simulink library "controls_element_lib"  (R2018b)
settings: Solver=VariableStepAuto  StartTime=0.0  StopTime=10.0  RelTol=1e-3
undefined symbols (not defined in the file): F_NOM, I_INV_BASE, j, P_INV_NOM, S_INV_NOM, S_NOM, S_PLANT, VHV_NOM, VLL_INV_NOM, VLL_NOM, Z_INV_BASE
libraries: simulink x20, $bdroot x5
(part 2 of 2)

== system controls_element_lib/acMonitor_A/SOGI ==
  in : Inport
  fnom : Inport  Port=2
  2pi : Gain  Gain=2*pi
  Integrator2 : Integrator
  Integrator3 : Integrator
  Product : Product
  Product1 : Product
  Sum4 : Sum  Inputs=|+-
  Sum5 : Sum  Inputs=|+-
  alpha : Gain  Gain=1 / sqrt(2)
  notch : Outport
  bpf : Outport  Port=2
  wires:
  in/1 -> Sum5/1
  fnom/1 -> 2pi/1
  Integrator2/1 -> Product1/1, Sum5/2, bpf/1
  alpha/1 -> Sum4/1
  Sum5/1 -> alpha/1, notch/1
  Sum4/1 -> Product/1
  Integrator3/1 -> Sum4/2
  2pi/1 -> Product1/2, Product/2
  Product/1 -> Integrator2/1
  Product1/1 -> Integrator3/1

== system controls_element_lib/circuitControls_B (SST)/virtual damper ==
  v : Inport
  1/tau_damp : Gain  Gain=1/250e-6
  Integrator : Integrator
  Sum : Sum  Inputs=|+-
  g_damp : Gain  Gain=1/(0.8*Z_INV_BASE)
  i_damp : Outport
  wires:
  1/tau_damp/1 -> Integrator/1
  Integrator/1 -> Sum/2
  v/1 -> Sum/1
  Sum/1 -> 1/tau_damp/1, g_damp/1
  g_damp/1 -> i_damp/1

== system controls_element_lib/circuit_controls_A/LPF ==
  1 : Inport
  Gain2 : Gain  Gain=1/20e-6
  Integrator : Integrator
  Sum4 : Sum  Inputs=|+-
  Out1 : Outport
  wires:
  Sum4/1 -> Gain2/1
  1/1 -> Sum4/1
  Integrator/1 -> Out1/1, Sum4/2
  Gain2/1 -> Integrator/1

== system controls_element_lib/circuit_controls_A/LPF1 ==
  1 : Inport
  Gain2 : Gain  Gain=1/20e-6
  Integrator : Integrator
  Sum4 : Sum  Inputs=|+-
  Out1 : Outport
  wires:
  Sum4/1 -> Gain2/1
  1/1 -> Sum4/1
  Integrator/1 -> Out1/1, Sum4/2
  Gain2/1 -> Integrator/1

== system controls_element_lib/circuit_controls_A/LPF2 ==
  1 : Inport
  Gain2 : Gain  Gain=1/20e-6
  Integrator : Integrator
  Sum4 : Sum  Inputs=|+-
  Out1 : Outport
  wires:
  Gain2/1 -> Integrator/1
  Integrator/1 -> Sum4/2, Out1/1
  1/1 -> Sum4/1
  Sum4/1 -> Gain2/1

== system controls_element_lib/circuit_controls_A/virtual damper ==
  v : Inport
  1/tau_damp : Gain  Gain=1/250e-6
  Integrator : Integrator
  Sum : Sum  Inputs=|+-
  g_damp : Gain  Gain=1/(0.8*Z_INV_BASE)
  i_damp : Outport
  wires:
  1/tau_damp/1 -> Integrator/1
  Integrator/1 -> Sum/2
  v/1 -> Sum/1
  Sum/1 -> 1/tau_damp/1, g_damp/1
  g_damp/1 -> i_damp/1

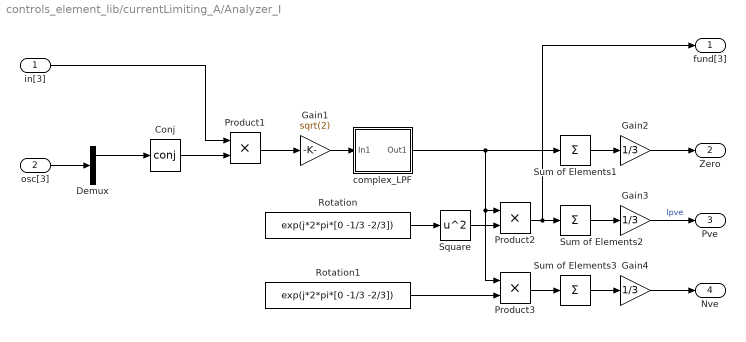
== system controls_element_lib/currentLimiting_A/Analyzer_I ==
  in[3] : Inport
  osc[3] : Inport  Port=2
  Conj : Math  Operator=conj  SaturateOnIntegerOverflow=on
  Demux : Demux  Outputs=3
  Gain1 : Gain  Gain=sqrt(2)
  Gain2 : Gain  Gain=1/3
  Gain3 : Gain  Gain=1/3
  Gain4 : Gain  Gain=1/3
  Product1 : Product
  Product2 : Product
  Product3 : Product
  Rotation : Constant  Value=exp(j*2*pi*[0 -1/3 -2/3])
  Rotation1 : Constant  Value=exp(j*2*pi*[0 -1/3 -2/3])
  Square : Math  Operator=square  SaturateOnIntegerOverflow=on
  Sum of Elements1 : Sum  Inputs=+
  Sum of Elements2 : Sum  Inputs=+
  Sum of Elements3 : Sum  Inputs=+
  complex_LPF : Subsystem  mask{tau=0.02}
      mask prompts: tau "Time constant"
  fund[3] : Outport
  Zero : Outport  Port=2
  Pve : Outport  Port=3
  Nve : Outport  Port=4
  wires:
  in[3]/1 -> Product1/1
  Gain2/1 -> Zero/1
  Gain3/1 -> Pve/1  "Ipve"
  osc[3]/1 -> Demux/1
  Sum of Elements3/1 -> Gain4/1
  Square/1 -> Product2/2
  Sum of Elements1/1 -> Gain2/1
  Conj/1 -> Product1/2
  Sum of Elements2/1 -> Gain3/1
  Rotation1/1 -> Product3/2
  Rotation/1 -> Square/1
  Demux/1 -> Conj/1
  Gain1/1 -> complex_LPF/1(In1)
  Product3/1 -> Sum of Elements3/1
  Product1/1 -> Gain1/1
  complex_LPF/1(Out1) -> Sum of Elements1/1, Product2/1, Product3/1
  Product2/1 -> Sum of Elements2/1, fund[3]/1
  Gain4/1 -> Nve/1

== system controls_element_lib/currentLimiting_A/excess_sink ==
  I_total[3] : Inport
  osc[3] : Inport  Port=2
  Irms_limit : Inport  Port=3
  Complex to Real-Imag : ComplexToRealImag
  Product3 : Product
  RMS Limiter : Subsystem
  Sum : Sum  Inputs=|-+
  sqrt(2) : Gain  Gain=sqrt(2)
  i_excess[3] : Outport
  wires:
  sqrt(2)/1 -> Product3/2
  Product3/1 -> Complex to Real-Imag/1
  I_total[3]/1 -> RMS Limiter/2(I[3]), Sum/2
  Sum/1 -> Product3/1  "Iexcess[3]"
  Complex to Real-Imag/1 -> i_excess[3]/1
  osc[3]/1 -> sqrt(2)/1
  Irms_limit/1 -> RMS Limiter/1(limit)
  RMS Limiter/1(I_limited[3]) -> Sum/1

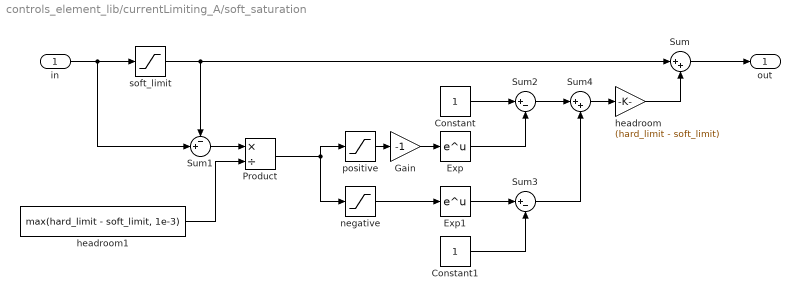
== system controls_element_lib/currentLimiting_A/soft_saturation ==
  in : Inport
  Constant : Constant
  Constant1 : Constant
  Exp : Math  SaturateOnIntegerOverflow=on
  Exp1 : Math  SaturateOnIntegerOverflow=on
  Gain : Gain  Gain=-1
  Product : Product  Inputs=*/
  Sum : Sum  Inputs=|++
  Sum1 : Sum  Inputs=-+|
  Sum2 : Sum  Inputs=|+-
  Sum3 : Sum  Inputs=|+-
  Sum4 : Sum  Inputs=|++
  headroom : Gain  Gain=(hard_limit - soft_limit)
  headroom1 : Constant  Value=max(hard_limit - soft_limit, 1e-3)
  negative : Saturate  UpperLimit=0  LowerLimit=-inf
  positive : Saturate  UpperLimit=inf  LowerLimit=0
  soft_limit : Saturate  UpperLimit=soft_limit  LowerLimit=-soft_limit
  out : Outport
  wires:
  Constant/1 -> Sum2/1
  Product/1 -> negative/1, positive/1
  Constant1/1 -> Sum3/2
  negative/1 -> Exp1/1
  Sum3/1 -> Sum4/2
  soft_limit/1 -> Sum/1, Sum1/1
  Sum/1 -> out/1
  Exp1/1 -> Sum3/1
  in/1 -> Sum1/2, soft_limit/1
  positive/1 -> Gain/1
  Exp/1 -> Sum2/2
  headroom/1 -> Sum/2
  Gain/1 -> Exp/1
  Sum4/1 -> headroom/1
  Sum2/1 -> Sum4/1
  Sum1/1 -> Product/1
  headroom1/1 -> Product/2

== system controls_element_lib/currentLimiting_B/RMS_Analyzer ==
  in : Inport
  Gain : Gain  Gain=1/0.02
  Integrator : Integrator
  Sqrt : Sqrt  SaturateOnIntegerOverflow=on
  Square : Math  Operator=square  SaturateOnIntegerOverflow=on
  Sum : Sum  Inputs=|+-
  RMS : Outport
  wires:
  Sqrt/1 -> RMS/1
  Integrator/1 -> Sqrt/1, Sum/2
  Sum/1 -> Gain/1
  Gain/1 -> Integrator/1
  in/1 -> Square/1
  Square/1 -> Sum/1

== system controls_element_lib/currentLimiting_B/SOGI_BPF ==
  in : Inport
  f : Inport  Port=2
  Gain : Gain
  Gain2 : Gain  Gain=2*pi
  Integrator : Integrator
  Integrator1 : Integrator
  Product : Product
  Product2 : Product
  Sum : Sum  Inputs=|+-
  Sum1 : Sum  Inputs=|+-
  bpf : Outport
  wires:
  Product2/1 -> Sum/2
  Sum/1 -> Product/1
  Gain2/1 -> Product/2, Product2/2
  Integrator/1 -> bpf/1, Gain/1, Integrator1/1
  Sum1/1 -> Sum/1
  Gain/1 -> Sum1/2
  Integrator1/1 -> Product2/1
  Product/1 -> Integrator/1
  in/1 -> Sum1/1
  f/1 -> Gain2/1

== system controls_element_lib/currentLimiting_B/estimate_excess ==
  Ilimit : Inport
  I[3] : Inport  Port=2
  Abs1 : Abs
  Constant : Constant
  Max : MinMax  Function=max
  Min : MinMax  Function=max  Inputs=2
  Product1 : Product  Inputs=*/
  Sum : Sum  Inputs=|+-
  excess_fraction : Outport
  wires:
  Min/1 -> Product1/2
  I[3]/1 -> Abs1/1
  Abs1/1 -> Max/1
  Ilimit/1 -> Min/1, Product1/1  "Irms_limit"
  Max/1 -> Min/2  "max_Iph"
  Product1/1 -> Sum/2  "scale_factor"
  Constant/1 -> Sum/1
  Sum/1 -> excess_fraction/1

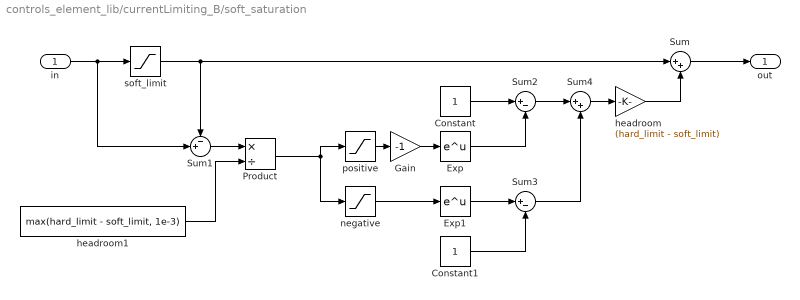
== system controls_element_lib/currentLimiting_B/soft_saturation ==
  in : Inport
  Constant : Constant
  Constant1 : Constant
  Exp : Math  SaturateOnIntegerOverflow=on
  Exp1 : Math  SaturateOnIntegerOverflow=on
  Gain : Gain  Gain=-1
  Product : Product  Inputs=*/
  Sum : Sum  Inputs=|++
  Sum1 : Sum  Inputs=-+|
  Sum2 : Sum  Inputs=|+-
  Sum3 : Sum  Inputs=|+-
  Sum4 : Sum  Inputs=|++
  headroom : Gain  Gain=(hard_limit - soft_limit)
  headroom1 : Constant  Value=max(hard_limit - soft_limit, 1e-3)
  negative : Saturate  UpperLimit=0  LowerLimit=-inf
  positive : Saturate  UpperLimit=inf  LowerLimit=0
  soft_limit : Saturate  UpperLimit=soft_limit  LowerLimit=-soft_limit
  out : Outport
  wires:
  Constant/1 -> Sum2/1
  Product/1 -> negative/1, positive/1
  Constant1/1 -> Sum3/2
  negative/1 -> Exp1/1
  Sum3/1 -> Sum4/2
  soft_limit/1 -> Sum/1, Sum1/1
  Sum/1 -> out/1
  Exp1/1 -> Sum3/1
  in/1 -> Sum1/2, soft_limit/1
  positive/1 -> Gain/1
  Exp/1 -> Sum2/2
  headroom/1 -> Sum/2
  Gain/1 -> Exp/1
  Sum4/1 -> headroom/1
  Sum2/1 -> Sum4/1
  Sum1/1 -> Product/1
  headroom1/1 -> Product/2

== system controls_element_lib/currentSource_A/current_modulator ==
  I_cmd : Inport
  osc : Inport  Port=2
  Complex to Real-Imag : ComplexToRealImag
  Complex to Real-Imag1 : ComplexToRealImag
  Gain : Gain  Gain=sqrt(2)
  Product1 : Product
  Product2 : Product
  Sum1 : Sum  Inputs=|+-
  i_ref : Outport
  wires:
  Complex to Real-Imag1/2 -> Product1/1
  Complex to Real-Imag1/1 -> Product2/1
  I_cmd/1 -> Complex to Real-Imag1/1
  Product1/1 -> Sum1/2
  Complex to Real-Imag/2 -> Product1/2
  Gain/1 -> Complex to Real-Imag/1
  Sum1/1 -> i_ref/1  "i"
  Product2/1 -> Sum1/1
  Complex to Real-Imag/1 -> Product2/2
  osc/1 -> Gain/1

== system controls_element_lib/dcVoltageRegulator_A/SOGI ==
  in : Inport
  fnom : Inport  Port=2
  2pi : Gain  Gain=2*pi
  Integrator2 : Integrator
  Integrator3 : Integrator
  Product : Product
  Product1 : Product
  Sum4 : Sum  Inputs=|+-
  Sum5 : Sum  Inputs=|+-
  alpha : Gain  Gain=1/sqrt(2)
  notch : Outport
  bpf : Outport  Port=2
  wires:
  in/1 -> Sum5/1
  fnom/1 -> 2pi/1
  Integrator2/1 -> Product1/1, Sum5/2, bpf/1
  alpha/1 -> Sum4/1
  Sum5/1 -> alpha/1, notch/1
  Sum4/1 -> Product/1
  Integrator3/1 -> Sum4/2
  2pi/1 -> Product1/2, Product/2
  Product/1 -> Integrator2/1
  Product1/1 -> Integrator3/1

== system controls_element_lib/machineModel_A/excitation ==
  note: This limit is needed to avoid excessive currents during blackstart that cause windup in current limiting logic.. It results in a linear ramp of voltage during blackstart
  VRef : Inport
  osc[3] : Inport  Port=2
  Vd : Inport  Port=3
  Complex to Real-Imag : ComplexToRealImag
  Gain2 : Gain  Gain=1/sqrt(3)
  LPF : TransferFcn  Denominator=[1/wExciter 1]
  Min : MinMax  Inputs=2
  Product1 : Product
  Saturation1 : Saturate  UpperLimit=1.1*VllRated  LowerLimit=0.9*VllRated
  Sum : Sum  Inputs=++|
  assymmetric filter1 : Subsystem
  sqrt(2) : Gain  Gain=sqrt(2)
  voltage_headroom : Constant  Value=0.3*VllRated
  v_emf : Outport
  wires:
  Vd/1 -> assymmetric filter1/1(in)  "Vd"
  assymmetric filter1/1(out) -> Sum/2  "Vd_conditioned"
  Product1/1 -> sqrt(2)/1
  Complex to Real-Imag/1 -> Product1/2
  osc[3]/1 -> Complex to Real-Imag/1
  Gain2/1 -> Product1/1  "Vref_LN"
  sqrt(2)/1 -> v_emf/1
  VRef/1 -> Saturation1/1  "VRef"
  Min/1 -> LPF/1
  LPF/1 -> Gain2/1  "Vref_LL"
  voltage_headroom/1 -> Sum/1
  Saturation1/1 -> Min/1
  Sum/1 -> Min/2

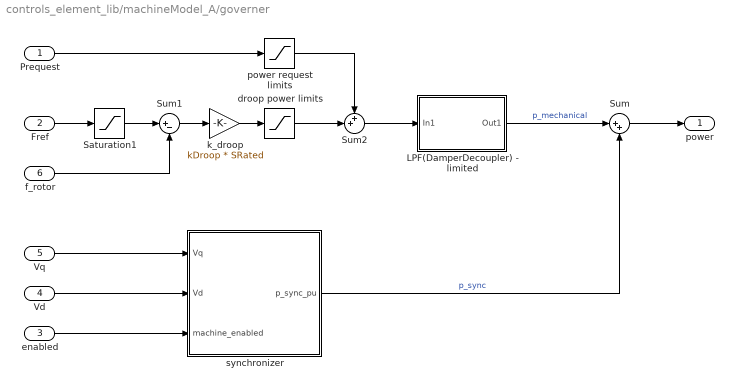
== system controls_element_lib/machineModel_A/governer ==
  Prequest : Inport
  Fref : Inport  Port=2
  enabled : Inport  Port=3
  Vd : Inport  Port=4
  Vq : Inport  Port=5
  f_rotor : Inport  Port=6
  LPF(DamperDecoupler) - limited : Subsystem
  Saturation1 : Saturate  UpperLimit=nominalFrequency+1  LowerLimit=nominalFrequency-1
  Sum : Sum  Inputs=|++
  Sum1 : Sum  Inputs=|+-
  Sum2 : Sum  Inputs=++|
  droop power limits : Saturate  UpperLimit=SRated  LowerLimit=-SRated
  k_droop : Gain  Gain=kDroop * SRated
  power request limits : Saturate  UpperLimit=SRated  LowerLimit=-SRated
  synchronizer : Subsystem
  power : Outport
  wires:
  Vd/1 -> synchronizer/2(Vd)
  Sum1/1 -> k_droop/1
  Sum/1 -> power/1
  Fref/1 -> Saturation1/1
  f_rotor/1 -> Sum1/2
  Saturation1/1 -> Sum1/1
  LPF(DamperDecoupler) - limited/1(Out1) -> Sum/1  "p_mechanical"
  enabled/1 -> synchronizer/3(machine_enabled)
  Sum2/1 -> LPF(DamperDecoupler) - limited/1(In1)
  k_droop/1 -> droop power limits/1
  Prequest/1 -> power request limits/1
  Vq/1 -> synchronizer/1(Vq)
  synchronizer/1(p_sync_pu) -> Sum/2  "p_sync"
  droop power limits/1 -> Sum2/2
  power request limits/1 -> Sum2/1

== system controls_element_lib/machineModel_A/impedance emulation ==
  v_emf : Inport
  enable : Inport  Port=2
  v_terminal : Inport  Port=3
  Constant : Constant  Value=0
  Integrator : Integrator
  Sum : Sum  Inputs=|+-
  Sum of Elements1 : Sum  Inputs=+
  Sum1 : Sum  Inputs=|+-
  Sum4 : Sum  Inputs=|+-
  Switch : Switch  Criteria=u2 > Threshold
  overLs : Gain  Gain=2*pi*60/(Xs * (VllRated^2/SRated))
  rN : Gain  Gain=0.2*(VllRated^2/SRated)
  rs : Gain  Gain=rs*(VllRated^2/SRated)
  i_ref : Outport
  wires:
  Integrator/1 -> i_ref/1, rs/1, Sum of Elements1/1  "i_ref"
  rs/1 -> Sum1/2
  rN/1 -> Sum4/2
  Sum1/1 -> overLs/1
  Sum4/1 -> Sum1/1
  Sum of Elements1/1 -> rN/1
  overLs/1 -> Integrator/1
  v_emf/1 -> Sum/1
  v_terminal/1 -> Sum/2
  Switch/1 -> Sum4/1
  Sum/1 -> Switch/1
  Constant/1 -> Switch/3
  enable/1 -> Switch/2

== system controls_element_lib/machineModel_A/power analyzer ==
  iac : Inport
  vac : Inport  Port=2
  Demux1 : Demux  Outputs=3
  Demux2 : Demux  Outputs=3
  Gain3 : Gain  Gain=1 / sqrt(3)
  Product{,1..3} (4 alike) : Product
  Sum of Elements : Sum  Inputs=+
  Sum2 : Sum  Inputs=|+-
  Sum3 : Sum  Inputs=|+-
  Sum4 : Sum  Inputs=|+-
  Sum5 : Sum  Inputs=+++
  P : Outport
  Q : Outport  Port=2
  wires:
  Product1/1 -> Sum5/1
  Product2/1 -> Sum5/3
  Sum4/1 -> Product3/1  "vca"
  Product3/1 -> Sum5/2
  Demux2/2 -> Sum3/1, Sum2/2
  Demux2/3 -> Sum4/1, Sum3/2
  Demux1/3 -> Product1/2  "ic"
  Demux1/2 -> Product3/2  "ib"
  vac/1 -> Demux2/1, Product/2
  iac/1 -> Product/1, Demux1/1
  Sum3/1 -> Product2/1  "vbc"
  Sum5/1 -> Gain3/1
  Sum2/1 -> Product1/1  "vab"
  Demux2/1 -> Sum4/2, Sum2/1
  Demux1/1 -> Product2/2  "ia"
  Gain3/1 -> Q/1  "Q"
  Sum of Elements/1 -> P/1  "P"
  Product/1 -> Sum of Elements/1

== system controls_element_lib/machineModel_A/rotor model ==
  p_mechanical : Inport
  p_electrical : Inport  Port=2
  Constant : Constant  Value=nominalFrequency
  HPF (wDamperDecoupler) : TransferFcn  Numerator=[0.3 0]  Denominator=[0.3 1]
  Integrator1 : Integrator  LimitOutput=on  UpperSaturationLimit=5  LowerSaturationLimit=-5
  Sum : Sum  Inputs=++|
  Sum2 : Sum  Inputs=|+-
  Sum3 : Sum  Inputs=|+-
  k_damp : Gain  Gain=kDamper*SRated
  k_inertia : Gain  Gain=(nominalFrequency/2)/(inertialConstant*SRated)
  oscillator_3ph : Subsystem
  osc[3] : Outport
  f_rotor : Outport  Port=2
  wires:
  Sum2/1 -> k_inertia/1
  k_inertia/1 -> Integrator1/1
  oscillator_3ph/1(osc[3]) -> osc[3]/1
  HPF (wDamperDecoupler)/1 -> k_damp/1
  p_electrical/1 -> Sum3/2
  Sum3/1 -> Sum2/1
  p_mechanical/1 -> Sum3/1
  Integrator1/1 -> Sum/2, HPF (wDamperDecoupler)/1
  k_damp/1 -> Sum2/2
  Sum/1 -> f_rotor/1, oscillator_3ph/1(f)
  Constant/1 -> Sum/1

== system controls_element_lib/machineModel_A/voltage analyzer ==
  osc[3] : Inport
  v_terminal : Inport  Port=2
  Complex to Real-Imag : ComplexToRealImag
  Conj : Math  Operator=conj  SaturateOnIntegerOverflow=on
  Product1 : Product
  Product2 : Product
  Sum of Elements1 : Sum  Inputs=+
  Sum of Elements2 : Sum  Inputs=+
  Transfer Fcn : TransferFcn  Denominator=[0.02 1]
  Transfer Fcn1 : TransferFcn  Denominator=[0.02 1]
  over_sqrt(3) : Gain  Gain=1/sqrt(3)
  over_sqrt(3)1 : Gain  Gain=1/sqrt(3)
  sqrt(2) : Gain  Gain=sqrt(2)
  Vd : Outport
  Vq : Outport  Port=2
  wires:
  Product2/1 -> Sum of Elements2/1
  Conj/1 -> sqrt(2)/1
  sqrt(2)/1 -> Complex to Real-Imag/1
  Sum of Elements1/1 -> over_sqrt(3)/1
  Product1/1 -> Sum of Elements1/1
  v_terminal/1 -> Product1/2, Product2/2
  Sum of Elements2/1 -> over_sqrt(3)1/1
  Complex to Real-Imag/2 -> Product1/1
  Complex to Real-Imag/1 -> Product2/1
  over_sqrt(3)/1 -> Transfer Fcn/1
  over_sqrt(3)1/1 -> Transfer Fcn1/1
  Transfer Fcn1/1 -> Vd/1  "Vd"
  osc[3]/1 -> Conj/1
  Transfer Fcn/1 -> Vq/1  "Vq"

== system controls_element_lib/modesAndProtection_A/hardware_protection ==
  vdc : Inport
  Clear Timer : Subsystem  mask{T_STEP=1e-3, TIMEOUT=dcTripClearTimeout}
      mask prompts: T_STEP "Time step"
  Compare To Constant1 : simulink/Logic and Bit Operations/Compare To Constant  relop=<  const=dcUndervotlageThreshold  OutDataTypeStr=boolean
  Compare To Constant2 : simulink/Logic and Bit Operations/Compare To Constant  relop=>  const=dcOvervotlageThreshold  OutDataTypeStr=boolean
  NOT : Logic  Operator=NOT  IconShape=distinctive  AllPortsSameDT=off  OutDataTypeStr=boolean
  OR : Logic  Operator=OR  IconShape=distinctive  AllPortsSameDT=off  OutDataTypeStr=boolean
  Zero-Order Hold1 : ZeroOrderHold  SampleTime=200e-6
  all_clear : Outport
  wires:
  vdc/1 -> Zero-Order Hold1/1
  Compare To Constant1/1 -> OR/2  "dcUV"
  OR/1 -> Clear Timer/1(in)
  Clear Timer/1(out) -> NOT/1
  Compare To Constant2/1 -> OR/1  "dcOV"
  Zero-Order Hold1/1 -> Compare To Constant1/1, Compare To Constant2/1
  NOT/1 -> all_clear/1

== system controls_element_lib/Battery plant controller/Meter/PLL-analog ==
  ref : Inport
  Gain : Gain  Gain=3
  Gain2 : Gain  Gain=30
  Integrator : Integrator  LimitOutput=on  UpperSaturationLimit=5  LowerSaturationLimit=-5
  Product2 : Product
  Real-Imag to Complex : RealImagToComplex
  Saturation : Saturate  UpperLimit=5  LowerLimit=-5
  Sum of Elements : Sum  Inputs=+
  Sum1 : Sum  Inputs=|-+
  Sum2 : Sum  Inputs=|++
  Transfer Fcn : TransferFcn  Denominator=[0.02 1]
  fnom : Constant  Value=60
  oscillator : Subsystem
  freq : Outport
  osc : Outport  Port=2
  wires:
  Sum of Elements/1 -> Transfer Fcn/1
  Real-Imag to Complex/1 -> osc/1
  oscillator/1(re) -> Real-Imag to Complex/1
  ref/1 -> Product2/1
  Sum1/1 -> oscillator/1(f), freq/1
  Gain/1 -> Saturation/1
  Saturation/1 -> Sum2/1
  Transfer Fcn/1 -> Gain2/1, Gain/1
  oscillator/2(im) -> Real-Imag to Complex/2, Product2/2
  Product2/1 -> Sum of Elements/1
  fnom/1 -> Sum1/2
  Sum2/1 -> Sum1/1
  Integrator/1 -> Sum2/2
  Gain2/1 -> Integrator/1

== system controls_element_lib/Datacenter plant controller/Meter/PLL-analog ==
  ref : Inport
  Gain : Gain  Gain=3
  Gain2 : Gain  Gain=30
  Integrator : Integrator  LimitOutput=on  UpperSaturationLimit=5  LowerSaturationLimit=-5
  Product2 : Product
  Real-Imag to Complex : RealImagToComplex
  Saturation : Saturate  UpperLimit=5  LowerLimit=-5
  Sum of Elements : Sum  Inputs=+
  Sum1 : Sum  Inputs=|-+
  Sum2 : Sum  Inputs=|++
  Transfer Fcn : TransferFcn  Denominator=[0.02 1]
  fnom : Constant  Value=60
  oscillator : Subsystem
  freq : Outport
  osc : Outport  Port=2
  wires:
  Sum of Elements/1 -> Transfer Fcn/1
  Real-Imag to Complex/1 -> osc/1
  oscillator/1(re) -> Real-Imag to Complex/1
  ref/1 -> Product2/1
  Sum1/1 -> oscillator/1(f), freq/1
  Gain/1 -> Saturation/1
  Saturation/1 -> Sum2/1
  Transfer Fcn/1 -> Gain2/1, Gain/1
  oscillator/2(im) -> Real-Imag to Complex/2, Product2/2
  Product2/1 -> Sum of Elements/1
  fnom/1 -> Sum1/2
  Sum2/1 -> Sum1/1
  Integrator/1 -> Sum2/2
  Gain2/1 -> Integrator/1

== system controls_element_lib/PV plant controller/Meter/PLL-analog ==
  ref : Inport
  Gain : Gain  Gain=3
  Gain2 : Gain  Gain=30
  Integrator : Integrator  LimitOutput=on  UpperSaturationLimit=5  LowerSaturationLimit=-5
  Product2 : Product
  Real-Imag to Complex : RealImagToComplex
  Saturation : Saturate  UpperLimit=5  LowerLimit=-5
  Sum of Elements : Sum  Inputs=+
  Sum1 : Sum  Inputs=|-+
  Sum2 : Sum  Inputs=|++
  Transfer Fcn : TransferFcn  Denominator=[0.02 1]
  fnom : Constant  Value=60
  oscillator : Subsystem
  freq : Outport
  osc : Outport  Port=2
  wires:
  Sum of Elements/1 -> Transfer Fcn/1
  Real-Imag to Complex/1 -> osc/1
  oscillator/1(re) -> Real-Imag to Complex/1
  ref/1 -> Product2/1
  Sum1/1 -> oscillator/1(f), freq/1
  Gain/1 -> Saturation/1
  Saturation/1 -> Sum2/1
  Transfer Fcn/1 -> Gain2/1, Gain/1
  oscillator/2(im) -> Real-Imag to Complex/2, Product2/2
  Product2/1 -> Sum of Elements/1
  fnom/1 -> Sum1/2
  Sum2/1 -> Sum1/1
  Integrator/1 -> Sum2/2
  Gain2/1 -> Integrator/1

== system controls_element_lib/acMonitor_A/Analyzer_V/complex_LPF ==
  note: This was needed because Simulink complains when using transfer functions directly on arrays or complex numbers.
  In1 : Inport
  Complex to Real-Imag : ComplexToRealImag
  Gain2 : Gain  Gain=1/tau
  Gain3 : Gain  Gain=1/tau
  Integrator : Integrator
  Integrator1 : Integrator
  Real-Imag to Complex : RealImagToComplex
  Sum : Sum  Inputs=|+-
  Sum1 : Sum  Inputs=|+-
  Out1 : Outport
  wires:
  Gain3/1 -> Integrator1/1
  Integrator1/1 -> Real-Imag to Complex/2, Sum1/2
  Sum/1 -> Gain2/1
  Gain2/1 -> Integrator/1
  Complex to Real-Imag/2 -> Sum1/1
  Sum1/1 -> Gain3/1
  Integrator/1 -> Sum/2, Real-Imag to Complex/1
  Complex to Real-Imag/1 -> Sum/1
  In1/1 -> Complex to Real-Imag/1
  Real-Imag to Complex/1 -> Out1/1

== system controls_element_lib/acMonitor_A/PLL_3ph/oscillator_3ph ==
  f : Inport
  Cos : Trigonometry  Operator=cos
  Gain : Gain  Gain=2*pi
  Integrator : Integrator
  Real-Imag to Complex : RealImagToComplex
  Sin : Trigonometry
  Sum1 : Sum  Inputs=|++
  phase_shift : Constant  Value=[0 -1/3 -2/3]
  osc[3] : Outport
  wires:
  f/1 -> Integrator/1
  Real-Imag to Complex/1 -> osc[3]/1
  Cos/1 -> Real-Imag to Complex/1
  Gain/1 -> Cos/1, Sin/1
  Integrator/1 -> Sum1/1
  Sin/1 -> Real-Imag to Complex/2
  phase_shift/1 -> Sum1/2
  Sum1/1 -> Gain/1

== system controls_element_lib/currentLimiting_A/Analyzer_I/complex_LPF ==
  note: This was needed because Simulink complains when using transfer functions directly on arrays or complex numbers.
  In1 : Inport
  Complex to Real-Imag : ComplexToRealImag
  Gain2 : Gain  Gain=1/tau
  Gain3 : Gain  Gain=1/tau
  Integrator : Integrator
  Integrator1 : Integrator
  Real-Imag to Complex : RealImagToComplex
  Sum : Sum  Inputs=|+-
  Sum1 : Sum  Inputs=|+-
  Out1 : Outport
  wires:
  Real-Imag to Complex/1 -> Out1/1
  In1/1 -> Complex to Real-Imag/1
  Complex to Real-Imag/1 -> Sum/1
  Integrator/1 -> Real-Imag to Complex/1, Sum/2
  Sum1/1 -> Gain3/1
  Complex to Real-Imag/2 -> Sum1/1
  Gain2/1 -> Integrator/1
  Sum/1 -> Gain2/1
  Integrator1/1 -> Sum1/2, Real-Imag to Complex/2
  Gain3/1 -> Integrator1/1

== system controls_element_lib/currentLimiting_A/excess_sink/RMS Limiter ==
  limit : Inport
  I[3] : Inport  Port=2
  Abs1 : Abs
  Max : MinMax  Function=max
  Min : MinMax  Function=max  Inputs=2
  Product1 : Product  Inputs=*/
  Product2 : Product
  I_limited[3] : Outport
  wires:
  Product2/1 -> I_limited[3]/1
  Min/1 -> Product1/2
  Max/1 -> Min/2  "highest phase current"
  Product1/1 -> Product2/1  "scale_factor"
  Abs1/1 -> Max/1
  I[3]/1 -> Product2/2, Abs1/1
  limit/1 -> Product1/1, Min/1

== system controls_element_lib/machineModel_A/excitation/assymmetric filter1 ==
  note: The saturation block is configured to cause a rapid rise, but much slow drop in output.
  in : Inport
  Gain1 : Gain  Gain=2
  Integrator : Integrator
  Saturation1 : Saturate  UpperLimit=VllRated  LowerLimit=-0.02 * VllRated
  Sum3 : Sum  Inputs=|+-
  out : Outport
  wires:
  Integrator/1 -> out/1, Sum3/2
  Sum3/1 -> Gain1/1
  in/1 -> Sum3/1
  Gain1/1 -> Saturation1/1
  Saturation1/1 -> Integrator/1

== system controls_element_lib/machineModel_A/governer/LPF(DamperDecoupler) - limited ==
  In1 : Inport
  Integrator : Integrator  LimitOutput=on  UpperSaturationLimit=1.2*SRated  LowerSaturationLimit=-1.2*SRated
  Sum3 : Sum  Inputs=|+-
  wDamperDecoupler : Gain  Gain=1/0.3
  Out1 : Outport
  wires:
  In1/1 -> Sum3/1
  wDamperDecoupler/1 -> Integrator/1
  Sum3/1 -> wDamperDecoupler/1
  Integrator/1 -> Sum3/2, Out1/1

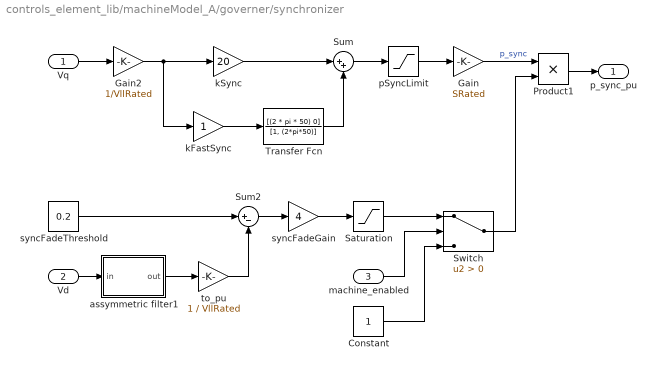
== system controls_element_lib/machineModel_A/governer/synchronizer ==
  Vq : Inport
  Vd : Inport  Port=2
  machine_enabled : Inport  Port=3
  Constant : Constant
  Gain : Gain  Gain=SRated
  Gain2 : Gain  Gain=1/VllRated
  Product1 : Product
  Saturation : Saturate  UpperLimit=1  LowerLimit=0
  Sum : Sum  Inputs=|++
  Sum2 : Sum  Inputs=|+-
  Switch : Switch  Criteria=u2 > Threshold
  Transfer Fcn : TransferFcn  Numerator=[(2 * pi * 50) 0]  Denominator=[1, (2*pi*50)]
  assymmetric filter1 : Subsystem
  kFastSync : Gain
  kSync : Gain  Gain=20
  pSyncLimit : Saturate  UpperLimit=3  LowerLimit=-3
  syncFadeGain : Gain  Gain=4
  syncFadeThreshold : Constant  Value=0.2
  to_pu : Gain  Gain=1 / VllRated
  p_sync_pu : Outport
  wires:
  Transfer Fcn/1 -> Sum/2
  Gain/1 -> Product1/1  "p_sync"
  Vq/1 -> Gain2/1
  Gain2/1 -> kSync/1, kFastSync/1
  Switch/1 -> Product1/2
  syncFadeThreshold/1 -> Sum2/1
  Saturation/1 -> Switch/1
  syncFadeGain/1 -> Saturation/1
  machine_enabled/1 -> Switch/2
  Sum2/1 -> syncFadeGain/1
  Constant/1 -> Switch/3
  Product1/1 -> p_sync_pu/1
  Sum/1 -> pSyncLimit/1
  kSync/1 -> Sum/1
  kFastSync/1 -> Transfer Fcn/1
  pSyncLimit/1 -> Gain/1
  assymmetric filter1/1(out) -> to_pu/1
  Vd/1 -> assymmetric filter1/1(in)
  to_pu/1 -> Sum2/2

== system controls_element_lib/machineModel_A/rotor model/oscillator_3ph ==
  f : Inport
  Cos : Trigonometry  Operator=cos
  Gain : Gain  Gain=2*pi
  Integrator : Integrator
  Real-Imag to Complex : RealImagToComplex
  Sin : Trigonometry
  Sum1 : Sum  Inputs=|++
  phase_shift : Constant  Value=[0 -1/3 -2/3]
  osc[3] : Outport
  wires:
  Sum1/1 -> Gain/1
  phase_shift/1 -> Sum1/2
  Sin/1 -> Real-Imag to Complex/2
  Integrator/1 -> Sum1/1
  Gain/1 -> Sin/1, Cos/1
  Cos/1 -> Real-Imag to Complex/1
  Real-Imag to Complex/1 -> osc[3]/1
  f/1 -> Integrator/1

== system controls_element_lib/modesAndProtection_A/hardware_protection/Clear Timer ==
  in : Inport
  Constant : Constant  Value=T_STEP
  Constant1 : Constant  Value=0
  Constant2 : Constant  Value=TIMEOUT
  Min2 : MinMax  Function=max  Inputs=2
  Relational Operator : RelationalOperator  Operator=>  OutDataTypeStr=boolean  RndMeth=Simplest
  Sum2 : Sum  Inputs=|-+
  Switch : Switch  Criteria=u2 > Threshold
  Unit Delay : UnitDelay  SampleTime=T_STEP  HasFrameUpgradeWarning=on
  out : Outport
  wires:
  Sum2/1 -> Relational Operator/1, Min2/1
  Constant1/1 -> Min2/2, Relational Operator/2
  Constant/1 -> Sum2/1
  Min2/1 -> Switch/3
  Constant2/1 -> Switch/1
  Unit Delay/1 -> Sum2/2
  in/1 -> Switch/2
  Switch/1 -> Unit Delay/1
  Relational Operator/1 -> out/1

== system controls_element_lib/Battery plant controller/Meter/PLL-analog/oscillator ==
  f : Inport
  2*pi : Gain  Gain=2*pi
  Cos : Trigonometry  Operator=cos
  Integrator : Integrator
  Rotation : Constant  Value=[0 -1 -2]*1/3
  Sin : Trigonometry
  Sum : Sum  Inputs=|++
  re : Outport
  im : Outport  Port=2
  wires:
  Rotation/1 -> Sum/2
  Integrator/1 -> Sum/1
  Sum/1 -> 2*pi/1
  Sin/1 -> im/1
  Cos/1 -> re/1
  f/1 -> Integrator/1
  2*pi/1 -> Cos/1, Sin/1

== system controls_element_lib/Datacenter plant controller/Meter/PLL-analog/oscillator ==
  f : Inport
  2*pi : Gain  Gain=2*pi
  Cos : Trigonometry  Operator=cos
  Integrator : Integrator
  Rotation : Constant  Value=[0 -1 -2]*1/3
  Sin : Trigonometry
  Sum : Sum  Inputs=|++
  re : Outport
  im : Outport  Port=2
  wires:
  Rotation/1 -> Sum/2
  Integrator/1 -> Sum/1
  Sum/1 -> 2*pi/1
  Sin/1 -> im/1
  Cos/1 -> re/1
  f/1 -> Integrator/1
  2*pi/1 -> Cos/1, Sin/1

== system controls_element_lib/PV plant controller/Meter/PLL-analog/oscillator ==
  f : Inport
  2*pi : Gain  Gain=2*pi
  Cos : Trigonometry  Operator=cos
  Integrator : Integrator
  Rotation : Constant  Value=[0 -1 -2]*1/3
  Sin : Trigonometry
  Sum : Sum  Inputs=|++
  re : Outport
  im : Outport  Port=2
  wires:
  Rotation/1 -> Sum/2
  Integrator/1 -> Sum/1
  Sum/1 -> 2*pi/1
  Sin/1 -> im/1
  Cos/1 -> re/1
  f/1 -> Integrator/1
  2*pi/1 -> Cos/1, Sin/1

== system controls_element_lib/machineModel_A/governer/synchronizer/assymmetric filter1 ==
  note: The saturation block is configured to cause a rapid rise, but much slow drop in output.
  in : Inport
  Gain1 : Gain  Gain=2
  Integrator : Integrator
  Saturation1 : Saturate  UpperLimit=VllRated  LowerLimit=-0.02 * VllRated
  Sum3 : Sum  Inputs=|+-
  out : Outport
  wires:
  Saturation1/1 -> Integrator/1
  Gain1/1 -> Saturation1/1
  in/1 -> Sum3/1
  Sum3/1 -> Gain1/1
  Integrator/1 -> Sum3/2, out/1
